simulink model "rlQuadrupedRobot"  (R2024b)
settings: Solver=ode23tb  StartTime=0.0  StopTime=10.0  RelTol=1e-3
values from neighbouring files (symbols this model uses):
  friction_force_max = mu_static * normal_force_max    [initializeRobotParameters.m]
  g = -9.81    [initializeRobotParameters.m]
  h_final = 0.75    [initializeRobotParameters.m]
  hip_eq_angle = 0    [initializeRobotParameters.m]
  init_ang_FL = d2r * quadrupedInverseKinematics(init_foot_disp_x,-init_body_height,l1,l2)    [initializeRobotParameters.m]
  init_ang_FR = init_ang_FL    [initializeRobotParameters.m]
  init_ang_RL = init_ang_FL    [initializeRobotParameters.m]
  init_ang_RR = init_ang_FL    [initializeRobotParameters.m]
  knee_eq_angle = 0    [initializeRobotParameters.m]
  l1 = 0.5517    [initializeRobotParameters.m]
  l2 = 0.5517    [initializeRobotParameters.m]
  L_back = 1.5    [initializeRobotParameters.m]
  M = 2    [initializeRobotParameters.m]
  m1 = 0.2    [initializeRobotParameters.m]
  m2 = 0.2    [initializeRobotParameters.m]
  normal_force_max = ((M+4*m1+4*m2)*abs(g))/4    [initializeRobotParameters.m]
  pitch_max = 10 * d2r    (= 0.174532925199)    [initializeRobotParameters.m]
  q_hip_max = -30 * d2r    (= -0.523598775598)    [initializeRobotParameters.m]
  q_hip_min = -120 * d2r    (= -2.09439510239)    [initializeRobotParameters.m]
  q_knee_max = 140 * d2r    (= 2.44346095279)    [initializeRobotParameters.m]
  q_knee_min = 60 * d2r    (= 1.0471975512)    [initializeRobotParameters.m]
  roll_max = 10 * d2r    (= 0.174532925199)    [initializeRobotParameters.m]
  Tf = 10    [initializeRobotParameters.m]
  Ts = 0.025    [initializeRobotParameters.m]
  u_max = 10    [initializeRobotParameters.m]
  vx_max = 2.5    [initializeRobotParameters.m]
  vy_max = 2.5    [initializeRobotParameters.m]
  vz_max = 2.5    [initializeRobotParameters.m]
  w_max = 2*pi*60/60    (= 6.28318530718)    [initializeRobotParameters.m]
  y_max = l1*cos(q_hip_max) + l2*cos(q_hip_max+q_knee_min)    [initializeRobotParameters.m]
  y_min = 0.5    [initializeRobotParameters.m]
  yaw_max = 20 * d2r    (= 0.349065850399)    [initializeRobotParameters.m]
  z_max = 0.5    [initializeRobotParameters.m]
undefined symbols (not defined in the file or in its folder): Extr_Data_LinkEndHole, Extr_Data_Mesh, ground, joint, X, Y, Z
libraries: sm_lib x113, nesl_utility x43, simulink x4, rllib x1
(part 2 of 5)

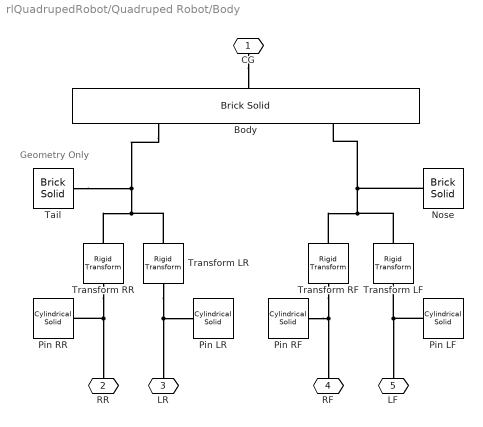
== system rlQuadrupedRobot/Quadruped Robot/Body ==
  note: Geometry Only
  Body : sm_lib/Body Elements/Brick Solid  BrickDimensions=[1 0.1 0.1]*L_back  BrickDimensionsUnits=m  ExportEntireGeometry=off  InertiaType=Custom  BasedOnType=Density  Density=1000  DensityUnits=kg/m^3  Mass=M  MassUnits=kg  CenterOfMass=[0 0 0]  CenterOfMassUnits=m  MomentsOfInertia=torso_MOI  MomentsOfInertiaUnits=kg*m^2  ProductsOfInertia=[1 1 1]*0  ProductsOfInertiaUnits=kg*m^2  GraphicType=FromGeometry  MarkerShape=Sphere  MarkerSize=10  GraphicVisPropType=SimpleVisualProperties  GraphicDiffuseColor=[164 184 200]/255  GraphicOpacity=1.0  GraphicSpecularColor=[0.5 0.5 0.5 1.0]  GraphicAmbientColor=[0.15 0.15 0.15 1.0]  GraphicEmissiveColor=[0.0 0.0 0.0 1.0]  GraphicShininess=75  DoExposeReferenceFrame=on  SerializedFrames=<Frames><Frame><Id>Frame1</Id><Value><Name>B</Name><Origin><Source>GeometricFeature</Source><FeatureName>-x surface</FeatureName></Origin><PrimaryAxis><DefinedDirection>+Z</DefinedDirection><Source>ReferenceFrame</Source><SourceDirection>+Z</SourceDirection><FeatureName></FeatureName></PrimaryAxis><SecondaryAxis><DefinedDirection>+X</DefinedDirection><Source>ReferenceFrame</Source><SourceDirection>+X</SourceDirection><FeatureName></FeatureName></SecondaryAxis></Value></Frame><Frame><Id>Frame2</Id><Value><Name>F</Name><Origin><Source>GeometricFeature</Source><FeatureName>+x surface</FeatureName></Origin><PrimaryAxis><DefinedDirection>+Z</DefinedDirection><Source>ReferenceFrame</Source><SourceDirection>+Z</SourceDirection><FeatureName></FeatureName></PrimaryAxis><SecondaryAxis><DefinedDirection>+X</DefinedDirection><Source>ReferenceFrame</Source><SourceDirection>+X</SourceDirection><FeatureName></FeatureName></SecondaryAxis></Value></Frame></Frames>
  Nose : sm_lib/Body Elements/Brick Solid  BrickDimensions=[0.05 0.1 0.1]*L_back  BrickDimensionsUnits=m  ExportEntireGeometry=off  InertiaType=CalculateFromGeometry  BasedOnType=Density  Density=0  DensityUnits=kg/m^3  Mass=1  MassUnits=kg  CenterOfMass=[0 0 0]  CenterOfMassUnits=m  MomentsOfInertia=[1 1 1]  MomentsOfInertiaUnits=kg*m^2  ProductsOfInertia=[1 1 1]  ProductsOfInertiaUnits=kg*m^2  GraphicType=FromGeometry  MarkerShape=Sphere  MarkerSize=10  GraphicVisPropType=SimpleVisualProperties  GraphicDiffuseColor=[164 184 200]/255  GraphicOpacity=1.0  GraphicSpecularColor=[0.5 0.5 0.5 1.0]  GraphicAmbientColor=[0.15 0.15 0.15 1.0]  GraphicEmissiveColor=[0.0 0.0 0.0 1.0]  GraphicShininess=75  DoExposeReferenceFrame=off  SerializedFrames=<Frames><Frame><Id>Frame1</Id><Value><Name>B</Name><Origin><Source>GeometricFeature</Source><FeatureName>-x surface</FeatureName></Origin><PrimaryAxis><DefinedDirection>+Z</DefinedDirection><Source>ReferenceFrame</Source><SourceDirection>+Z</SourceDirection><FeatureName></FeatureName></PrimaryAxis><SecondaryAxis><DefinedDirection>+X</DefinedDirection><Source>ReferenceFrame</Source><SourceDirection>+X</SourceDirection><FeatureName></FeatureName></SecondaryAxis></Value></Frame></Frames>
  Pin LF : sm_lib/Body Elements/Cylindrical Solid  CylinderRadius=0.025*l1  CylinderRadiusUnits=m  CylinderLength=0.1*l1  CylinderLengthUnits=m  ExportEntireGeometry=off  InertiaType=CalculateFromGeometry  BasedOnType=Density  Density=0  DensityUnits=kg/m^3  Mass=1  MassUnits=kg  CenterOfMass=[0 0 0]  CenterOfMassUnits=m  MomentsOfInertia=[1 1 1]  MomentsOfInertiaUnits=kg*m^2  ProductsOfInertia=[1 1 1]  ProductsOfInertiaUnits=kg*m^2  GraphicType=FromGeometry  MarkerShape=Sphere  MarkerSize=10  GraphicVisPropType=SimpleVisualProperties  GraphicDiffuseColor=[164 184 200]/255  GraphicOpacity=1.0  GraphicSpecularColor=[0.5 0.5 0.5 1.0]  GraphicAmbientColor=[0.15 0.15 0.15 1.0]  GraphicEmissiveColor=[0.0 0.0 0.0 1.0]  GraphicShininess=75  DoExposeReferenceFrame=off  SerializedFrames=<Frames><Frame><Id>Frame1</Id><Value><Name>F</Name><Origin><Source>GeometricFeature</Source><FeatureName>top surface</FeatureName></Origin><PrimaryAxis><DefinedDirection>+Z</DefinedDirection><Source>ReferenceFrame</Source><SourceDirection>+Z</SourceDirection><FeatureName></FeatureName></PrimaryAxis><SecondaryAxis><DefinedDirection>+X</DefinedDirection><Source>ReferenceFrame</Source><SourceDirection>+X</SourceDirection><FeatureName></FeatureName></SecondaryAxis></Value></Frame><Frame><Id>Frame2</Id><Value><Name>B</Name><Origin><Source>GeometricFeature</Source><FeatureName>bottom surface</FeatureName></Origin><PrimaryAxis><DefinedDirection>+Z</DefinedDirection><Source>ReferenceFrame</Source><SourceDirection>+Z</SourceDirection><FeatureName></FeatureName></PrimaryAxis><SecondaryAxis><DefinedDirection>+X</DefinedDirection><Source>ReferenceFrame</Source><SourceDirection>+X</SourceDirection><FeatureName></FeatureName></SecondaryAxis></Value></Frame></Frames>
  Pin LR : sm_lib/Body Elements/Cylindrical Solid  CylinderRadius=0.025*l1  CylinderRadiusUnits=m  CylinderLength=0.1*l1  CylinderLengthUnits=m  ExportEntireGeometry=off  InertiaType=CalculateFromGeometry  BasedOnType=Density  Density=0  DensityUnits=kg/m^3  Mass=1  MassUnits=kg  CenterOfMass=[0 0 0]  CenterOfMassUnits=m  MomentsOfInertia=[1 1 1]  MomentsOfInertiaUnits=kg*m^2  ProductsOfInertia=[1 1 1]  ProductsOfInertiaUnits=kg*m^2  GraphicType=FromGeometry  MarkerShape=Sphere  MarkerSize=10  GraphicVisPropType=SimpleVisualProperties  GraphicDiffuseColor=[164 184 200]/255  GraphicOpacity=1.0  GraphicSpecularColor=[0.5 0.5 0.5 1.0]  GraphicAmbientColor=[0.15 0.15 0.15 1.0]  GraphicEmissiveColor=[0.0 0.0 0.0 1.0]  GraphicShininess=75  DoExposeReferenceFrame=off  SerializedFrames=<Frames><Frame><Id>Frame1</Id><Value><Name>F</Name><Origin><Source>GeometricFeature</Source><FeatureName>top surface</FeatureName></Origin><PrimaryAxis><DefinedDirection>+Z</DefinedDirection><Source>ReferenceFrame</Source><SourceDirection>+Z</SourceDirection><FeatureName></FeatureName></PrimaryAxis><SecondaryAxis><DefinedDirection>+X</DefinedDirection><Source>ReferenceFrame</Source><SourceDirection>+X</SourceDirection><FeatureName></FeatureName></SecondaryAxis></Value></Frame><Frame><Id>Frame2</Id><Value><Name>B</Name><Origin><Source>GeometricFeature</Source><FeatureName>bottom surface</FeatureName></Origin><PrimaryAxis><DefinedDirection>+Z</DefinedDirection><Source>ReferenceFrame</Source><SourceDirection>+Z</SourceDirection><FeatureName></FeatureName></PrimaryAxis><SecondaryAxis><DefinedDirection>+X</DefinedDirection><Source>ReferenceFrame</Source><SourceDirection>+X</SourceDirection><FeatureName></FeatureName></SecondaryAxis></Value></Frame></Frames>
  Pin RF : sm_lib/Body Elements/Cylindrical Solid  CylinderRadius=0.025*l1  CylinderRadiusUnits=m  CylinderLength=0.1*l1  CylinderLengthUnits=m  ExportEntireGeometry=off  InertiaType=CalculateFromGeometry  BasedOnType=Density  Density=0  DensityUnits=kg/m^3  Mass=1  MassUnits=kg  CenterOfMass=[0 0 0]  CenterOfMassUnits=m  MomentsOfInertia=[1 1 1]  MomentsOfInertiaUnits=kg*m^2  ProductsOfInertia=[1 1 1]  ProductsOfInertiaUnits=kg*m^2  GraphicType=FromGeometry  MarkerShape=Sphere  MarkerSize=10  GraphicVisPropType=SimpleVisualProperties  GraphicDiffuseColor=[164 184 200]/255  GraphicOpacity=1.0  GraphicSpecularColor=[0.5 0.5 0.5 1.0]  GraphicAmbientColor=[0.15 0.15 0.15 1.0]  GraphicEmissiveColor=[0.0 0.0 0.0 1.0]  GraphicShininess=75  DoExposeReferenceFrame=off  SerializedFrames=<Frames><Frame><Id>Frame1</Id><Value><Name>F</Name><Origin><Source>GeometricFeature</Source><FeatureName>top surface</FeatureName></Origin><PrimaryAxis><DefinedDirection>+Z</DefinedDirection><Source>ReferenceFrame</Source><SourceDirection>+Z</SourceDirection><FeatureName></FeatureName></PrimaryAxis><SecondaryAxis><DefinedDirection>+X</DefinedDirection><Source>ReferenceFrame</Source><SourceDirection>+X</SourceDirection><FeatureName></FeatureName></SecondaryAxis></Value></Frame><Frame><Id>Frame2</Id><Value><Name>B</Name><Origin><Source>GeometricFeature</Source><FeatureName>bottom surface</FeatureName></Origin><PrimaryAxis><DefinedDirection>+Z</DefinedDirection><Source>ReferenceFrame</Source><SourceDirection>+Z</SourceDirection><FeatureName></FeatureName></PrimaryAxis><SecondaryAxis><DefinedDirection>+X</DefinedDirection><Source>ReferenceFrame</Source><SourceDirection>+X</SourceDirection><FeatureName></FeatureName></SecondaryAxis></Value></Frame></Frames>
  Pin RR : sm_lib/Body Elements/Cylindrical Solid  CylinderRadius=0.025*l1  CylinderRadiusUnits=m  CylinderLength=0.1*l1  CylinderLengthUnits=m  ExportEntireGeometry=off  InertiaType=CalculateFromGeometry  BasedOnType=Density  Density=0  DensityUnits=kg/m^3  Mass=1  MassUnits=kg  CenterOfMass=[0 0 0]  CenterOfMassUnits=m  MomentsOfInertia=[1 1 1]  MomentsOfInertiaUnits=kg*m^2  ProductsOfInertia=[1 1 1]  ProductsOfInertiaUnits=kg*m^2  GraphicType=FromGeometry  MarkerShape=Sphere  MarkerSize=10  GraphicVisPropType=SimpleVisualProperties  GraphicDiffuseColor=[164 184 200]/255  GraphicOpacity=1.0  GraphicSpecularColor=[0.5 0.5 0.5 1.0]  GraphicAmbientColor=[0.15 0.15 0.15 1.0]  GraphicEmissiveColor=[0.0 0.0 0.0 1.0]  GraphicShininess=75  DoExposeReferenceFrame=off  SerializedFrames=<Frames><Frame><Id>Frame1</Id><Value><Name>F</Name><Origin><Source>GeometricFeature</Source><FeatureName>top surface</FeatureName></Origin><PrimaryAxis><DefinedDirection>+Z</DefinedDirection><Source>ReferenceFrame</Source><SourceDirection>+Z</SourceDirection><FeatureName></FeatureName></PrimaryAxis><SecondaryAxis><DefinedDirection>+X</DefinedDirection><Source>ReferenceFrame</Source><SourceDirection>+X</SourceDirection><FeatureName></FeatureName></SecondaryAxis></Value></Frame><Frame><Id>Frame2</Id><Value><Name>B</Name><Origin><Source>GeometricFeature</Source><FeatureName>bottom surface</FeatureName></Origin><PrimaryAxis><DefinedDirection>+Z</DefinedDirection><Source>ReferenceFrame</Source><SourceDirection>+Z</SourceDirection><FeatureName></FeatureName></PrimaryAxis><SecondaryAxis><DefinedDirection>+X</DefinedDirection><Source>ReferenceFrame</Source><SourceDirection>+X</SourceDirection><FeatureName></FeatureName></SecondaryAxis></Value></Frame></Frames>
  Tail : sm_lib/Body Elements/Brick Solid  BrickDimensions=[0.05 0.1 0.1]*L_back  BrickDimensionsUnits=m  ExportEntireGeometry=off  InertiaType=CalculateFromGeometry  BasedOnType=Density  Density=0  DensityUnits=kg/m^3  Mass=1  MassUnits=kg  CenterOfMass=[0 0 0]  CenterOfMassUnits=m  MomentsOfInertia=[1 1 1]  MomentsOfInertiaUnits=kg*m^2  ProductsOfInertia=[1 1 1]  ProductsOfInertiaUnits=kg*m^2  GraphicType=FromGeometry  MarkerShape=Sphere  MarkerSize=10  GraphicVisPropType=SimpleVisualProperties  GraphicDiffuseColor=[164 184 200]/255  GraphicOpacity=1.0  GraphicSpecularColor=[0.5 0.5 0.5 1.0]  GraphicAmbientColor=[0.15 0.15 0.15 1.0]  GraphicEmissiveColor=[0.0 0.0 0.0 1.0]  GraphicShininess=75  DoExposeReferenceFrame=off  SerializedFrames=<Frames><Frame><Id>Frame1</Id><Value><Name>F</Name><Origin><Source>GeometricFeature</Source><FeatureName>+x surface</FeatureName></Origin><PrimaryAxis><DefinedDirection>+Z</DefinedDirection><Source>ReferenceFrame</Source><SourceDirection>+Z</SourceDirection><FeatureName></FeatureName></PrimaryAxis><SecondaryAxis><DefinedDirection>+X</DefinedDirection><Source>ReferenceFrame</Source><SourceDirection>+X</SourceDirection><FeatureName></FeatureName></SecondaryAxis></Value></Frame></Frames>
  Transform LF : sm_lib/Frames and Transforms/Rigid Transform  RotationMethod=None  FollAlignAxisA=+X  BaseAlignAxisA=+Y  FollAlignAxisB=+Y  BaseAlignAxisB=+Z  RotationStandardAxis=+Z  RotationAngle=0.0  RotationAngleUnits=deg  RotationArbitraryAxis=[0 0 1]  RotationSequenceAxes=FollowerAxes  RotationSequence=XYX  RotationSequenceAngles=[0 0 0]  RotationSequenceAnglesUnits=deg  RotationMatrix=[1 0 0; 0 1 0; 0 0 1]  Quaternion=[1 0 0 0]  TranslationMethod=StandardAxis  TranslationCartesianOffset=[0 0 0]  TranslationCartesianOffsetUnits=m  TranslationStandardAxis=+Z  TranslationStandardOffset=0.1*L_back/2  TranslationStandardOffsetUnits=m  TranslationROffset=0  TranslationROffsetUnits=m  TranslationThetaOffset=0  TranslationThetaOffsetUnits=deg  TranslationZOffset=0  TranslationZOffsetUnits=m
  Transform LR : sm_lib/Frames and Transforms/Rigid Transform  RotationMethod=None  FollAlignAxisA=+X  BaseAlignAxisA=+Y  FollAlignAxisB=+Y  BaseAlignAxisB=+Z  RotationStandardAxis=+Z  RotationAngle=0.0  RotationAngleUnits=deg  RotationArbitraryAxis=[0 0 1]  RotationSequenceAxes=FollowerAxes  RotationSequence=XYX  RotationSequenceAngles=[0 0 0]  RotationSequenceAnglesUnits=deg  RotationMatrix=[1 0 0; 0 1 0; 0 0 1]  Quaternion=[1 0 0 0]  TranslationMethod=StandardAxis  TranslationCartesianOffset=[0 0 0]  TranslationCartesianOffsetUnits=m  TranslationStandardAxis=+Z  TranslationStandardOffset=0.1*L_back/2  TranslationStandardOffsetUnits=m  TranslationROffset=0  TranslationROffsetUnits=m  TranslationThetaOffset=0  TranslationThetaOffsetUnits=deg  TranslationZOffset=0  TranslationZOffsetUnits=m
  Transform RF : sm_lib/Frames and Transforms/Rigid Transform  RotationMethod=None  FollAlignAxisA=+X  BaseAlignAxisA=+Y  FollAlignAxisB=+Y  BaseAlignAxisB=+Z  RotationStandardAxis=+Z  RotationAngle=0.0  RotationAngleUnits=deg  RotationArbitraryAxis=[0 0 1]  RotationSequenceAxes=FollowerAxes  RotationSequence=XYX  RotationSequenceAngles=[0 0 0]  RotationSequenceAnglesUnits=deg  RotationMatrix=[1 0 0; 0 1 0; 0 0 1]  Quaternion=[1 0 0 0]  TranslationMethod=StandardAxis  TranslationCartesianOffset=[0 0 0]  TranslationCartesianOffsetUnits=m  TranslationStandardAxis=+Z  TranslationStandardOffset=0.1*L_back/2  TranslationStandardOffsetUnits=m  TranslationROffset=0  TranslationROffsetUnits=m  TranslationThetaOffset=0  TranslationThetaOffsetUnits=deg  TranslationZOffset=0  TranslationZOffsetUnits=m
  Transform RR : sm_lib/Frames and Transforms/Rigid Transform  RotationMethod=None  FollAlignAxisA=+X  BaseAlignAxisA=+Y  FollAlignAxisB=+Y  BaseAlignAxisB=+Z  RotationStandardAxis=+Z  RotationAngle=0.0  RotationAngleUnits=deg  RotationArbitraryAxis=[0 0 1]  RotationSequenceAxes=FollowerAxes  RotationSequence=XYX  RotationSequenceAngles=[0 0 0]  RotationSequenceAnglesUnits=deg  RotationMatrix=[1 0 0; 0 1 0; 0 0 1]  Quaternion=[1 0 0 0]  TranslationMethod=StandardAxis  TranslationCartesianOffset=[0 0 0]  TranslationCartesianOffsetUnits=m  TranslationStandardAxis=+Z  TranslationStandardOffset=0.1*L_back/2  TranslationStandardOffsetUnits=m  TranslationROffset=0  TranslationROffsetUnits=m  TranslationThetaOffset=0  TranslationThetaOffsetUnits=deg  TranslationZOffset=0  TranslationZOffsetUnits=m
  CG : PMIOPort  Side=Right
  RR : PMIOPort  Port=2  Side=Left
  LR : PMIOPort  Port=3  Side=Left
  RF : PMIOPort  Port=4  Side=Left
  LF : PMIOPort  Port=5  Side=Left
  connections:
  Pin LF/RConn1 -- LF/RConn1 -- Transform LF/RConn1
  CG/RConn1 -- Body/RConn1
  Transform LF/LConn1 -- Transform RF/RConn1 -- Body/LConn2 -- Nose/LConn1
  Transform RF/LConn1 -- RF/RConn1 -- Pin RF/LConn1
  Body/LConn1 -- Tail/LConn1 -- Transform LR/LConn1 -- Transform RR/RConn1
  Transform RR/LConn1 -- Pin RR/LConn1 -- RR/RConn1
  Transform LR/RConn1 -- LR/RConn1 -- Pin LR/RConn1

== system rlQuadrupedRobot/Quadruped Robot/Floor ==
  Floor : sm_lib/Body Elements/Brick Solid  BrickDimensions=[100 0.05 1]  BrickDimensionsUnits=m  ExportEntireGeometry=on  InertiaType=CalculateFromGeometry  BasedOnType=Density  Density=1000  DensityUnits=kg/m^3  Mass=1  MassUnits=kg  CenterOfMass=[0 0 0]  CenterOfMassUnits=m  MomentsOfInertia=[1 1 1]  MomentsOfInertiaUnits=kg*m^2  ProductsOfInertia=[1 1 1]  ProductsOfInertiaUnits=kg*m^2  GraphicType=FromGeometry  MarkerShape=Sphere  MarkerSize=10  GraphicVisPropType=SimpleVisualProperties  GraphicDiffuseColor=[0.5 0.5 0.5]  GraphicOpacity=1.0  GraphicSpecularColor=[0.5 0.5 0.5 1.0]  GraphicAmbientColor=[0.15 0.15 0.15 1.0]  GraphicEmissiveColor=[0.0 0.0 0.0 1.0]  GraphicShininess=75  DoExposeReferenceFrame=on  SerializedFrames=<Frames/>
  Mechanism Configuration : sm_lib/Utilities/Mechanism Configuration  UniformGravity=Constant  GravityVector=[0 g 0]  GravityVectorUnits=m/s^2  LinearizationDelta=0.001  JointModeTransitionNonlinearIterations=2
  Mesh : sm_lib/Body Elements/Extruded Solid  ExtrusionType=General  PolygonNumSides=3  PolygonOuterRadius=1  PolygonOuterRadiusUnits=m  ExportEntireGeometry=off  ExtrusionCrossSection=Extr_Data_Mesh(100,1,100,1,0.9,0.9)  ExtrusionCrossSectionUnits=m  ExportConvexHullGeometry=off  ExtrusionLength=0.055  ExtrusionLengthUnits=m  InertiaType=CalculateFromGeometry  BasedOnType=Density  Density=1000  DensityUnits=kg/m^3  Mass=1  MassUnits=kg  CenterOfMass=[0 0 0]  CenterOfMassUnits=m  MomentsOfInertia=[1 1 1]  MomentsOfInertiaUnits=kg*m^2  ProductsOfInertia=[1 1 1]  ProductsOfInertiaUnits=kg*m^2  GraphicType=FromGeometry  MarkerShape=Sphere  MarkerSize=10  GraphicVisPropType=SimpleVisualProperties  GraphicDiffuseColor=[1.0 1.0 1.0]  GraphicOpacity=1.0  GraphicSpecularColor=[0.5 0.5 0.5 1.0]  GraphicAmbientColor=[0.15 0.15 0.15 1.0]  GraphicEmissiveColor=[0.0 0.0 0.0 1.0]  GraphicShininess=75  DoExposeReferenceFrame=on  SerializedFrames=<Frames/>
  Solver Configuration : nesl_utility/Solver Configuration  PhysicalDomain=network_engine_domain  SubClassName=solver  LeftPortType=input  RightPortType=generic  Tones=[]  Harmonics=[]  SimulateNoise=off  Profile=off  UseLocalSampling=off  EnableSwitchedLinearOptims=on  FrequencyDomain=off  UseCCode=off  RelTol=0.001  AbsTol=1e-06  MinStep=1e-09  ToWorkspace=off  RevertToSquareIcSolve=off  NumHomotopyIterations=100  PhasorMode=off  PhasorModeNumHarmonics=1  ConsistencySolver=NEWTON_FTOL  IndexReductionMethod=DerivativeReplacement  DoDC=off  ResidualTolerance=1e-9  ConsistencyTolSource=GLOBAL  ConsistencyAbsTol=0.001  ConsistencyRelTol=0.001  ConsistencyTolFactor=0.001  UseLocalSolver=off  LocalSolverChoice=NE_BACKWARD_EULER_ADVANCER  ResolveIndetEquations=on  FunctionEvalNumThread=1  LocalSolverSampleTime=.001  DoFixedCost=off  MaxNonlinIter=12  MaxModeIter=2  ComputeImpulses=off  ImpulseIterations=2  LinearAlgebra=Sparse  LinearAlgebraNumThread=0  EquationFormulation=NE_TIME_EF  DelaysMemoryBudget=1024  AutomaticFiltering=on  FilteringTimeConstant=0.001  PartitionStorageMethod=AS_NEEDED  PartitionMemoryBudget=1024  PartitionMethod=FAST  MultibodyUseLocalSolver=off  MultibodyLocalSolverChoice=ODE1  MultibodyLocalSolverSampleTime=0.001
  Transform Floor Frame : sm_lib/Frames and Transforms/Rigid Transform  RotationMethod=None  FollAlignAxisA=+X  BaseAlignAxisA=+Y  FollAlignAxisB=+Y  BaseAlignAxisB=+Z  RotationStandardAxis=+X  RotationAngle=-90  RotationAngleUnits=deg  RotationArbitraryAxis=[0 0 1]  RotationSequenceAxes=FollowerAxes  RotationSequence=XYX  RotationSequenceAngles=[0 0 0]  RotationSequenceAnglesUnits=deg  RotationMatrix=[1 0 0; 0 1 0; 0 0 1]  Quaternion=[1 0 0 0]  TranslationMethod=StandardAxis  TranslationCartesianOffset=[0 0 0]  TranslationCartesianOffsetUnits=m  TranslationStandardAxis=-Y  TranslationStandardOffset=0.056/2  TranslationStandardOffsetUnits=m  TranslationROffset=0  TranslationROffsetUnits=m  TranslationThetaOffset=0  TranslationThetaOffsetUnits=deg  TranslationZOffset=0  TranslationZOffsetUnits=m
  Transform Mesh : sm_lib/Frames and Transforms/Rigid Transform  RotationMethod=StandardAxis  FollAlignAxisA=+X  BaseAlignAxisA=+Y  FollAlignAxisB=+Y  BaseAlignAxisB=+Z  RotationStandardAxis=-X  RotationAngle=90  RotationAngleUnits=deg  RotationArbitraryAxis=[0 0 1]  RotationSequenceAxes=FollowerAxes  RotationSequence=XYX  RotationSequenceAngles=[0 0 0]  RotationSequenceAnglesUnits=deg  RotationMatrix=[1 0 0; 0 1 0; 0 0 1]  Quaternion=[1 0 0 0]  TranslationMethod=None  TranslationCartesianOffset=[0 0 0]  TranslationCartesianOffsetUnits=m  TranslationStandardAxis=+Z  TranslationStandardOffset=0  TranslationStandardOffsetUnits=m  TranslationROffset=0  TranslationROffsetUnits=m  TranslationThetaOffset=0  TranslationThetaOffsetUnits=deg  TranslationZOffset=0  TranslationZOffsetUnits=m
  World Frame : sm_lib/Frames and Transforms/World Frame
  FG : PMIOPort  Side=Right
  W : PMIOPort  Port=2  Side=Left
  connections:
  Mesh/RConn1 -- Transform Mesh/RConn1
  Floor/RConn1 -- Transform Mesh/LConn1 -- Transform Floor Frame/RConn1
  Transform Floor Frame/LConn1 -- World Frame/RConn1 -- Solver Configuration/RConn1 -- Mechanism Configuration/RConn1 -- W/RConn1
  FG/RConn1 -- Floor/LConn1

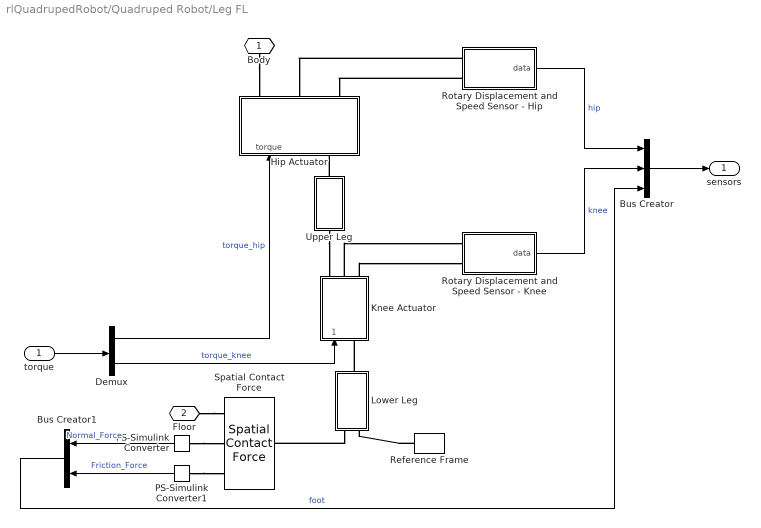
== system rlQuadrupedRobot/Quadruped Robot/Leg FL ==
  torque : Inport
  Bus Creator : BusCreator  Inputs=3
  Bus Creator1 : BusCreator  Inputs=2
  Demux : Demux  Outputs=2
  Hip Actuator : Subsystem
  Knee Actuator : Subsystem
  Lower Leg : Subsystem
  PS-Simulink Converter : nesl_utility/PS-Simulink Converter  PhysicalDomain=network_engine_domain  SubClassName=ps_output  LeftPortType=input  RightPortType=output  PseudoPeriodic=off  Frequencies=[]  VectorFormat=1-D array  Unit=inherit  AffineConversion=off
  PS-Simulink Converter1 : nesl_utility/PS-Simulink Converter  PhysicalDomain=network_engine_domain  SubClassName=ps_output  LeftPortType=input  RightPortType=output  PseudoPeriodic=off  Frequencies=[]  VectorFormat=1-D array  Unit=inherit  AffineConversion=off
  Reference Frame : sm_lib/Frames and Transforms/Reference Frame
  Rotary Displacement and Speed Sensor - Hip : Subsystem
  Rotary Displacement and Speed Sensor - Knee : Subsystem
  Spatial Contact Force : sm_lib/Forces and Torques/Spatial Contact Force  NormalForceType=SmoothSpringDamper  NormalStiffness=ground.stiffness  NormalStiffnessUnits=N/m  NormalDamping=ground.damping  NormalDampingUnits=N/(m/s)  NormalTransitionRegionWidth=ground.depth/2  NormalTransitionRegionWidthUnits=m  FrictionType=SmoothStickSlip  CoefficientOfStaticFriction=mu_static  CoefficientOfDynamicFriction=mu_kinetic  FrictionalCriticalVelocity=v_thres  FrictionalCriticalVelocityUnits=m/s  SenseContactSignal=off  SensePenetrationDepth=off  SenseSeparationDistance=off  SenseNormalForceMagnitude=on  SenseFrictionalForceMagnitude=on  SenseNormalVelocity=off  SenseTangentialVelocity=off  SenseContactBaseRotation=off  SenseContactBaseTranslation=off  SenseContactFollowerRotation=off  SenseContactFollowerTranslation=off  ZeroCrossDetectContactStartAndEnd=off
  Upper Leg : Subsystem
  Body : PMIOPort  Side=Left
  Floor : PMIOPort  Tag=PMCPort  Port=2  Side=Right
  sensors : Outport  VectorParamsAs1DForOutWhenUnconnected=off
  wires:
  Bus Creator/1 -> sensors/1
  Rotary Displacement and Speed Sensor - Knee/1(data) -> Bus Creator/2  "knee"
  Rotary Displacement and Speed Sensor - Hip/1(data) -> Bus Creator/1  "hip"
  Demux/2 -> Knee Actuator/1(torque)  "torque_knee"
  Demux/1 -> Hip Actuator/1(torque)  "torque_hip"
  torque/1 -> Demux/1
  PS-Simulink Converter1/1 -> Bus Creator1/2  "Friction_Force"
  PS-Simulink Converter/1 -> Bus Creator1/1  "Normal_Force"
  Bus Creator1/1 -> Bus Creator/3  "foot"
  connections:
  Knee Actuator/RConn3 -- Rotary Displacement and Speed Sensor - Knee/LConn2
  Knee Actuator/RConn2 -- Rotary Displacement and Speed Sensor - Knee/LConn1
  Rotary Displacement and Speed Sensor - Hip/LConn2 -- Hip Actuator/RConn3
  Rotary Displacement and Speed Sensor - Hip/LConn1 -- Hip Actuator/RConn2
  Upper Leg/LConn1 -- Knee Actuator/RConn1
  Upper Leg/RConn1 -- Hip Actuator/LConn1
  Lower Leg/RConn1 -- Knee Actuator/LConn1
  Body/RConn1 -- Hip Actuator/RConn1
  Lower Leg/LConn1 -- Spatial Contact Force/LConn1
  Floor/RConn1 -- Spatial Contact Force/RConn1
  PS-Simulink Converter1/LConn1 -- Spatial Contact Force/RConn3
  PS-Simulink Converter/LConn1 -- Spatial Contact Force/RConn2
  Reference Frame/RConn1 -- Lower Leg/LConn2

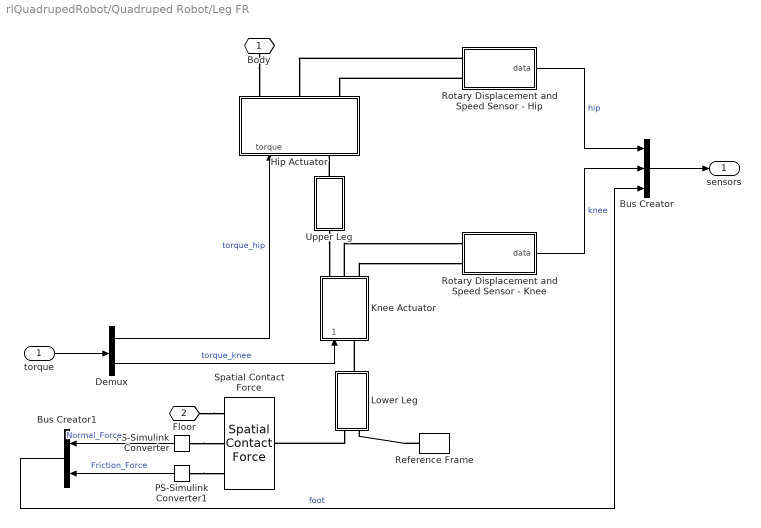
== system rlQuadrupedRobot/Quadruped Robot/Leg FR ==
  torque : Inport
  Bus Creator : BusCreator  Inputs=3
  Bus Creator1 : BusCreator  Inputs=2
  Demux : Demux  Outputs=2
  Hip Actuator : Subsystem
  Knee Actuator : Subsystem
  Lower Leg : Subsystem
  PS-Simulink Converter : nesl_utility/PS-Simulink Converter  PhysicalDomain=network_engine_domain  SubClassName=ps_output  LeftPortType=input  RightPortType=output  PseudoPeriodic=off  Frequencies=[]  VectorFormat=1-D array  Unit=inherit  AffineConversion=off
  PS-Simulink Converter1 : nesl_utility/PS-Simulink Converter  PhysicalDomain=network_engine_domain  SubClassName=ps_output  LeftPortType=input  RightPortType=output  PseudoPeriodic=off  Frequencies=[]  VectorFormat=1-D array  Unit=inherit  AffineConversion=off
  Reference Frame : sm_lib/Frames and Transforms/Reference Frame
  Rotary Displacement and Speed Sensor - Hip : Subsystem
  Rotary Displacement and Speed Sensor - Knee : Subsystem
  Spatial Contact Force : sm_lib/Forces and Torques/Spatial Contact Force  NormalForceType=SmoothSpringDamper  NormalStiffness=ground.stiffness  NormalStiffnessUnits=N/m  NormalDamping=ground.damping  NormalDampingUnits=N/(m/s)  NormalTransitionRegionWidth=ground.depth/2  NormalTransitionRegionWidthUnits=m  FrictionType=SmoothStickSlip  CoefficientOfStaticFriction=mu_static  CoefficientOfDynamicFriction=mu_kinetic  FrictionalCriticalVelocity=v_thres  FrictionalCriticalVelocityUnits=m/s  SenseContactSignal=off  SensePenetrationDepth=off  SenseSeparationDistance=off  SenseNormalForceMagnitude=on  SenseFrictionalForceMagnitude=on  SenseNormalVelocity=off  SenseTangentialVelocity=off  SenseContactBaseRotation=off  SenseContactBaseTranslation=off  SenseContactFollowerRotation=off  SenseContactFollowerTranslation=off  ZeroCrossDetectContactStartAndEnd=off
  Upper Leg : Subsystem
  Body : PMIOPort  Side=Left
  Floor : PMIOPort  Tag=PMCPort  Port=2  Side=Right
  sensors : Outport  VectorParamsAs1DForOutWhenUnconnected=off
  wires:
  Bus Creator/1 -> sensors/1
  Rotary Displacement and Speed Sensor - Knee/1(data) -> Bus Creator/2  "knee"
  Rotary Displacement and Speed Sensor - Hip/1(data) -> Bus Creator/1  "hip"
  Demux/2 -> Knee Actuator/1(torque)  "torque_knee"
  Demux/1 -> Hip Actuator/1(torque)  "torque_hip"
  torque/1 -> Demux/1
  PS-Simulink Converter1/1 -> Bus Creator1/2  "Friction_Force"
  PS-Simulink Converter/1 -> Bus Creator1/1  "Normal_Force"
  Bus Creator1/1 -> Bus Creator/3  "foot"
  connections:
  Knee Actuator/RConn3 -- Rotary Displacement and Speed Sensor - Knee/LConn2
  Knee Actuator/RConn2 -- Rotary Displacement and Speed Sensor - Knee/LConn1
  Rotary Displacement and Speed Sensor - Hip/LConn2 -- Hip Actuator/RConn3
  Rotary Displacement and Speed Sensor - Hip/LConn1 -- Hip Actuator/RConn2
  Upper Leg/LConn1 -- Knee Actuator/RConn1
  Upper Leg/RConn1 -- Hip Actuator/LConn1
  Lower Leg/RConn1 -- Knee Actuator/LConn1
  Body/RConn1 -- Hip Actuator/RConn1
  Lower Leg/LConn1 -- Spatial Contact Force/LConn1
  Floor/RConn1 -- Spatial Contact Force/RConn1
  PS-Simulink Converter1/LConn1 -- Spatial Contact Force/RConn3
  PS-Simulink Converter/LConn1 -- Spatial Contact Force/RConn2
  Reference Frame/RConn1 -- Lower Leg/LConn2

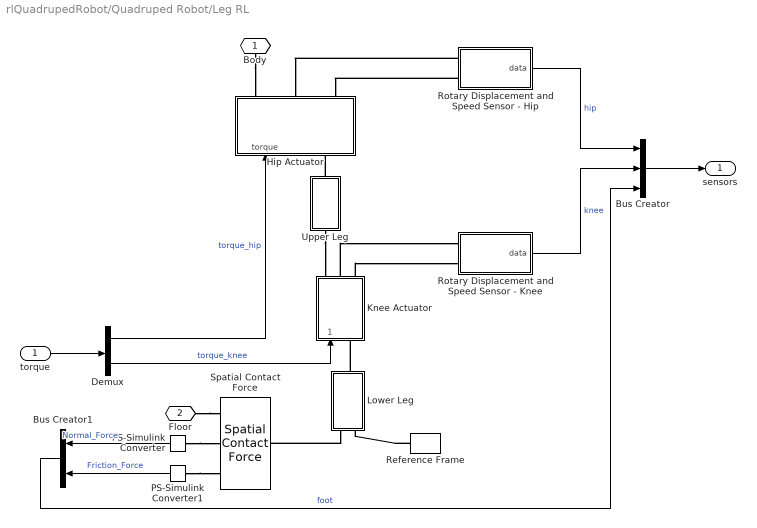
== system rlQuadrupedRobot/Quadruped Robot/Leg RL ==
  torque : Inport
  Bus Creator : BusCreator  Inputs=3
  Bus Creator1 : BusCreator  Inputs=2
  Demux : Demux  Outputs=2
  Hip Actuator : Subsystem
  Knee Actuator : Subsystem
  Lower Leg : Subsystem
  PS-Simulink Converter : nesl_utility/PS-Simulink Converter  PhysicalDomain=network_engine_domain  SubClassName=ps_output  LeftPortType=input  RightPortType=output  PseudoPeriodic=off  Frequencies=[]  VectorFormat=1-D array  Unit=inherit  AffineConversion=off
  PS-Simulink Converter1 : nesl_utility/PS-Simulink Converter  PhysicalDomain=network_engine_domain  SubClassName=ps_output  LeftPortType=input  RightPortType=output  PseudoPeriodic=off  Frequencies=[]  VectorFormat=1-D array  Unit=inherit  AffineConversion=off
  Reference Frame : sm_lib/Frames and Transforms/Reference Frame
  Rotary Displacement and Speed Sensor - Hip : Subsystem
  Rotary Displacement and Speed Sensor - Knee : Subsystem
  Spatial Contact Force : sm_lib/Forces and Torques/Spatial Contact Force  NormalForceType=SmoothSpringDamper  NormalStiffness=ground.stiffness  NormalStiffnessUnits=N/m  NormalDamping=ground.damping  NormalDampingUnits=N/(m/s)  NormalTransitionRegionWidth=ground.depth/2  NormalTransitionRegionWidthUnits=m  FrictionType=SmoothStickSlip  CoefficientOfStaticFriction=mu_static  CoefficientOfDynamicFriction=mu_kinetic  FrictionalCriticalVelocity=v_thres  FrictionalCriticalVelocityUnits=m/s  SenseContactSignal=off  SensePenetrationDepth=off  SenseSeparationDistance=off  SenseNormalForceMagnitude=on  SenseFrictionalForceMagnitude=on  SenseNormalVelocity=off  SenseTangentialVelocity=off  SenseContactBaseRotation=off  SenseContactBaseTranslation=off  SenseContactFollowerRotation=off  SenseContactFollowerTranslation=off  ZeroCrossDetectContactStartAndEnd=off
  Upper Leg : Subsystem
  Body : PMIOPort  Side=Left
  Floor : PMIOPort  Tag=PMCPort  Port=2  Side=Right
  sensors : Outport  VectorParamsAs1DForOutWhenUnconnected=off
  wires:
  Bus Creator/1 -> sensors/1
  Rotary Displacement and Speed Sensor - Knee/1(data) -> Bus Creator/2  "knee"
  Rotary Displacement and Speed Sensor - Hip/1(data) -> Bus Creator/1  "hip"
  Demux/2 -> Knee Actuator/1(torque)  "torque_knee"
  Demux/1 -> Hip Actuator/1(torque)  "torque_hip"
  torque/1 -> Demux/1
  PS-Simulink Converter1/1 -> Bus Creator1/2  "Friction_Force"
  PS-Simulink Converter/1 -> Bus Creator1/1  "Normal_Force"
  Bus Creator1/1 -> Bus Creator/3  "foot"
  connections:
  Knee Actuator/RConn3 -- Rotary Displacement and Speed Sensor - Knee/LConn2
  Knee Actuator/RConn2 -- Rotary Displacement and Speed Sensor - Knee/LConn1
  Rotary Displacement and Speed Sensor - Hip/LConn2 -- Hip Actuator/RConn3
  Rotary Displacement and Speed Sensor - Hip/LConn1 -- Hip Actuator/RConn2
  Upper Leg/LConn1 -- Knee Actuator/RConn1
  Upper Leg/RConn1 -- Hip Actuator/LConn1
  Lower Leg/RConn1 -- Knee Actuator/LConn1
  Body/RConn1 -- Hip Actuator/RConn1
  Lower Leg/LConn1 -- Spatial Contact Force/LConn1
  Floor/RConn1 -- Spatial Contact Force/RConn1
  PS-Simulink Converter1/LConn1 -- Spatial Contact Force/RConn3
  PS-Simulink Converter/LConn1 -- Spatial Contact Force/RConn2
  Reference Frame/RConn1 -- Lower Leg/LConn2

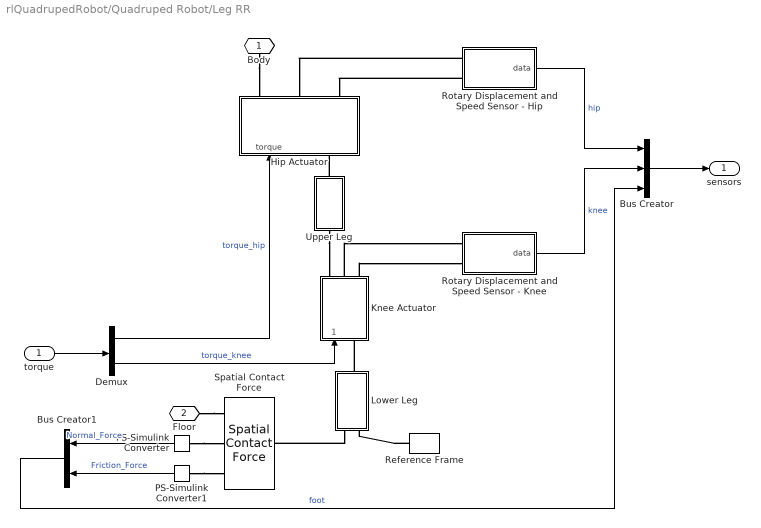
== system rlQuadrupedRobot/Quadruped Robot/Leg RR ==
  torque : Inport
  Bus Creator : BusCreator  Inputs=3
  Bus Creator1 : BusCreator  Inputs=2
  Demux : Demux  Outputs=2
  Hip Actuator : Subsystem
  Knee Actuator : Subsystem
  Lower Leg : Subsystem
  PS-Simulink Converter : nesl_utility/PS-Simulink Converter  PhysicalDomain=network_engine_domain  SubClassName=ps_output  LeftPortType=input  RightPortType=output  PseudoPeriodic=off  Frequencies=[]  VectorFormat=1-D array  Unit=inherit  AffineConversion=off
  PS-Simulink Converter1 : nesl_utility/PS-Simulink Converter  PhysicalDomain=network_engine_domain  SubClassName=ps_output  LeftPortType=input  RightPortType=output  PseudoPeriodic=off  Frequencies=[]  VectorFormat=1-D array  Unit=inherit  AffineConversion=off
  Reference Frame : sm_lib/Frames and Transforms/Reference Frame
  Rotary Displacement and Speed Sensor - Hip : Subsystem
  Rotary Displacement and Speed Sensor - Knee : Subsystem
  Spatial Contact Force : sm_lib/Forces and Torques/Spatial Contact Force  NormalForceType=SmoothSpringDamper  NormalStiffness=ground.stiffness  NormalStiffnessUnits=N/m  NormalDamping=ground.damping  NormalDampingUnits=N/(m/s)  NormalTransitionRegionWidth=ground.depth/2  NormalTransitionRegionWidthUnits=m  FrictionType=SmoothStickSlip  CoefficientOfStaticFriction=mu_static  CoefficientOfDynamicFriction=mu_kinetic  FrictionalCriticalVelocity=v_thres  FrictionalCriticalVelocityUnits=m/s  SenseContactSignal=off  SensePenetrationDepth=off  SenseSeparationDistance=off  SenseNormalForceMagnitude=on  SenseFrictionalForceMagnitude=on  SenseNormalVelocity=off  SenseTangentialVelocity=off  SenseContactBaseRotation=off  SenseContactBaseTranslation=off  SenseContactFollowerRotation=off  SenseContactFollowerTranslation=off  ZeroCrossDetectContactStartAndEnd=off
  Upper Leg : Subsystem
  Body : PMIOPort  Side=Left
  Floor : PMIOPort  Tag=PMCPort  Port=2  Side=Right
  sensors : Outport  VectorParamsAs1DForOutWhenUnconnected=off
  wires:
  Bus Creator/1 -> sensors/1
  Rotary Displacement and Speed Sensor - Knee/1(data) -> Bus Creator/2  "knee"
  Rotary Displacement and Speed Sensor - Hip/1(data) -> Bus Creator/1  "hip"
  Demux/2 -> Knee Actuator/1(torque)  "torque_knee"
  Demux/1 -> Hip Actuator/1(torque)  "torque_hip"
  torque/1 -> Demux/1
  Bus Creator1/1 -> Bus Creator/3  "foot"
  PS-Simulink Converter1/1 -> Bus Creator1/2  "Friction_Force"
  PS-Simulink Converter/1 -> Bus Creator1/1  "Normal_Force"
  connections:
  Floor/RConn1 -- Spatial Contact Force/RConn1
  Knee Actuator/RConn3 -- Rotary Displacement and Speed Sensor - Knee/LConn2
  Knee Actuator/RConn2 -- Rotary Displacement and Speed Sensor - Knee/LConn1
  Rotary Displacement and Speed Sensor - Hip/LConn2 -- Hip Actuator/RConn3
  Rotary Displacement and Speed Sensor - Hip/LConn1 -- Hip Actuator/RConn2
  Upper Leg/LConn1 -- Knee Actuator/RConn1
  Upper Leg/RConn1 -- Hip Actuator/LConn1
  Lower Leg/RConn1 -- Knee Actuator/LConn1
  Body/RConn1 -- Hip Actuator/RConn1
  Lower Leg/LConn1 -- Spatial Contact Force/LConn1
  PS-Simulink Converter/LConn1 -- Spatial Contact Force/RConn2
  PS-Simulink Converter1/LConn1 -- Spatial Contact Force/RConn3
  Reference Frame/RConn1 -- Lower Leg/LConn2

== system rlQuadrupedRobot/Quadruped Robot/Sensors ==
  Body Sensors : Subsystem
  Bus Creator : BusCreator  Inputs=5
  From : From  TagVisibility=global
  Leg Sensors : Subsystem
  Visualization Camera : Subsystem
  CG : PMIOPort  Side=Left
  W : PMIOPort  Port=2  Side=Left
  sensors_out : Outport  VectorParamsAs1DForOutWhenUnconnected=off
  wires:
  Body Sensors/1(bodyBus) -> Bus Creator/1  "body"
  Bus Creator/1 -> sensors_out/1
  From/1 -> Leg Sensors/1(FL)
  [B] -> Leg Sensors/2(FR)
  [C] -> Leg Sensors/3(RL)
  [D] -> Leg Sensors/4(RR)
  Leg Sensors/1(FLbus) -> Bus Creator/2  "leg_FL"
  Leg Sensors/2(FRbus) -> Bus Creator/3  "leg_FR"
  Leg Sensors/3(RLbus) -> Bus Creator/4  "leg_RL"
  Leg Sensors/4(RRbus) -> Bus Creator/5  "leg_RR"
  connections:
  Body Sensors/LConn2 -- W/RConn1
  Body Sensors/LConn1 -- Visualization Camera/LConn1 -- CG/RConn1

== system rlQuadrupedRobot/Quadruped Robot/Subsystem ==
  torques : Inport
  Demux : Demux  Outputs=8
  Mux{,1..3} (4 alike) : Mux  Inputs=2
  FL : Outport  VectorParamsAs1DForOutWhenUnconnected=off
  FR : Outport  Port=2  VectorParamsAs1DForOutWhenUnconnected=off
  RL : Outport  Port=3  VectorParamsAs1DForOutWhenUnconnected=off
  RR : Outport  Port=4  VectorParamsAs1DForOutWhenUnconnected=off
  wires:
  torques/1 -> Demux/1
  Demux/2 -> Mux/2  "torque_knee_FL"
  Demux/3 -> Mux1/1  "torque_hip_FR"
  Demux/4 -> Mux1/2  "torque_knee_FR"
  Demux/5 -> Mux2/1  "torque_hip_RL"
  Demux/6 -> Mux2/2  "torque_knee_RL"
  Demux/8 -> Mux3/2  "torque_knee_RR"
  Demux/7 -> Mux3/1  "torque_hip_RR"
  Mux/1 -> FL/1  "torque_FL"
  Mux1/1 -> FR/1  "torque_FR"
  Mux2/1 -> RL/1  "torque_RL"
  Mux3/1 -> RR/1  "torque_RR"
  Demux/1 -> Mux/1  "torque_hip_FL"

== system rlQuadrupedRobot/Quadruped Robot/Leg FL/Hip Actuator ==
  torque : Inport
  Revolute Hip : sm_lib/Joints/Revolute Joint  JointMode=Normal  CompositeWrenchDir=FollowerOnBase  CompositeWrenchFrame=BaseFrame  SenseConstraintForce=off  SenseConstraintTorque=off  SenseTotalForce=off  SenseTotalTorque=off  PositionTargetSpecify=on  PositionTargetPriority=High  PositionTargetValue=-th1_0  PositionTargetValueUnits=rad  VelocityTargetSpecify=on  VelocityTargetPriority=High  VelocityTargetValue=th1_dot_0  VelocityTargetValueUnits=rad/s  EquilibriumPosition=eqAngle_hip  EquilibriumPositionUnits=rad  SpringStiffness=k_hip  SpringStiffnessUnits=N*m/rad  DampingCoefficient=b_hip  DampingCoefficientUnits=N*m/(rad/s)  LowerLimitSpecify=on  LowerLimitBound=-q_hip_max  LowerLimitBoundUnits=rad  LowerLimitStiffness=klim_hip  LowerLimitStiffnessUnits=N*m/rad  LowerLimitDamping=blim_hip  LowerLimitDampingUnits=N*m/(rad/s)  LowerLimitTransitionRegionWidth=tr_width_hip  LowerLimitTransitionRegionWidthUnits=rad  UpperLimitSpecify=on  UpperLimitBound=-q_hip_min  UpperLimitBoundUnits=rad  UpperLimitStiffness=klim_hip  UpperLimitStiffnessUnits=N*m/rad  UpperLimitDamping=blim_hip  UpperLimitDampingUnits=N*m/(rad/s)  UpperLimitTransitionRegionWidth=tr_width_hip  UpperLimitTransitionRegionWidthUnits=rad  TorqueActuationMode=InputTorque  MotionActuationMode=ComputedMotion  SensePosition=on  SenseVelocity=on  SenseAcceleration=off  SenseTorqueForce=off  SenseLowerLimitTorqueForce=off  SenseUpperLimitTorqueForce=off
  Simulink-PS Converter : nesl_utility/Simulink-PS Converter  PhysicalDomain=network_engine_domain  SubClassName=ps_input  LeftPortType=input  RightPortType=output  PseudoPeriodic=off  Frequencies=[]  NoiseDistribution=none  NoiseParameters=[]  Unit=1  AffineConversion=off  FilteringAndDerivatives=provide  SimscapeFilterOrder=1  InputFilterTimeConstant=0.001  UdotUserProvided=0
  Transform Link : sm_lib/Frames and Transforms/Rigid Transform  RotationMethod=None  FollAlignAxisA=+X  BaseAlignAxisA=+Y  FollAlignAxisB=+Y  BaseAlignAxisB=+Z  RotationStandardAxis=+Z  RotationAngle=0.0  RotationAngleUnits=deg  RotationArbitraryAxis=[0 0 1]  RotationSequenceAxes=FollowerAxes  RotationSequence=XYX  RotationSequenceAngles=[0 0 0]  RotationSequenceAnglesUnits=deg  RotationMatrix=[1 0 0; 0 1 0; 0 0 1]  Quaternion=[1 0 0 0]  TranslationMethod=StandardAxis  TranslationCartesianOffset=[0 0 0]  TranslationCartesianOffsetUnits=m  TranslationStandardAxis=+Z  TranslationStandardOffset=leg_width*sideSign/2  TranslationStandardOffsetUnits=m  TranslationROffset=0  TranslationROffsetUnits=m  TranslationThetaOffset=0  TranslationThetaOffsetUnits=deg  TranslationZOffset=0  TranslationZOffsetUnits=m
  B : PMIOPort  Side=Left
  F : PMIOPort  Port=2  Side=Right
  q : PMIOPort  Port=3  Side=Right
  w : PMIOPort  Port=4  Side=Right
  wires:
  torque/1 -> Simulink-PS Converter/1
  connections:
  w/RConn1 -- Revolute Hip/RConn3
  Revolute Hip/RConn2 -- q/RConn1
  Simulink-PS Converter/RConn1 -- Revolute Hip/LConn2
  B/RConn1 -- Transform Link/LConn1
  F/RConn1 -- Revolute Hip/RConn1
  Transform Link/RConn1 -- Revolute Hip/LConn1

== system rlQuadrupedRobot/Quadruped Robot/Leg FL/Knee Actuator ==
  torque : Inport
  Revolute Knee : sm_lib/Joints/Revolute Joint  JointMode=Normal  CompositeWrenchDir=FollowerOnBase  CompositeWrenchFrame=BaseFrame  SenseConstraintForce=off  SenseConstraintTorque=off  SenseTotalForce=off  SenseTotalTorque=off  PositionTargetSpecify=on  PositionTargetPriority=High  PositionTargetValue=-th2_0  PositionTargetValueUnits=rad  VelocityTargetSpecify=on  VelocityTargetPriority=High  VelocityTargetValue=0  VelocityTargetValueUnits=rad/s  EquilibriumPosition=eqAngle_knee  EquilibriumPositionUnits=rad  SpringStiffness=k_knee  SpringStiffnessUnits=N*m/rad  DampingCoefficient=b_knee  DampingCoefficientUnits=N*m/(rad/s)  LowerLimitSpecify=on  LowerLimitBound=-q_knee_max  LowerLimitBoundUnits=rad  LowerLimitStiffness=klim_knee  LowerLimitStiffnessUnits=N*m/rad  LowerLimitDamping=blim_knee  LowerLimitDampingUnits=N*m/(rad/s)  LowerLimitTransitionRegionWidth=tr_width_knee  LowerLimitTransitionRegionWidthUnits=rad  UpperLimitSpecify=on  UpperLimitBound=-q_knee_min  UpperLimitBoundUnits=rad  UpperLimitStiffness=klim_knee  UpperLimitStiffnessUnits=N*m/rad  UpperLimitDamping=blim_knee  UpperLimitDampingUnits=N*m/(rad/s)  UpperLimitTransitionRegionWidth=tr_width_knee  UpperLimitTransitionRegionWidthUnits=rad  TorqueActuationMode=InputTorque  MotionActuationMode=ComputedMotion  SensePosition=on  SenseVelocity=on  SenseAcceleration=off  SenseTorqueForce=off  SenseLowerLimitTorqueForce=off  SenseUpperLimitTorqueForce=off
  Simulink-PS Converter : nesl_utility/Simulink-PS Converter  PhysicalDomain=network_engine_domain  SubClassName=ps_input  LeftPortType=input  RightPortType=output  PseudoPeriodic=off  Frequencies=[]  NoiseDistribution=none  NoiseParameters=[]  Unit=1  AffineConversion=off  FilteringAndDerivatives=provide  SimscapeFilterOrder=1  InputFilterTimeConstant=0.005  UdotUserProvided=0
  B : PMIOPort  Side=Left
  F : PMIOPort  Port=2  Side=Right
  q : PMIOPort  Port=3  Side=Right
  w : PMIOPort  Port=4  Side=Right
  wires:
  torque/1 -> Simulink-PS Converter/1
  connections:
  Revolute Knee/RConn3 -- w/RConn1
  q/RConn1 -- Revolute Knee/RConn2
  Revolute Knee/LConn1 -- B/RConn1
  Simulink-PS Converter/RConn1 -- Revolute Knee/LConn2
  F/RConn1 -- Revolute Knee/RConn1
